simulink model "Quadruped_view"  (R2026a)
settings: Solver=ode23tb  StopTime=50
values from neighbouring files (symbols this model uses):
  a_amp = 0.03    [initializeRobotParameters.m]
  b_amp = 0.03    [initializeRobotParameters.m]
  dTheta = 20*pi/180    (= 0.349065850399)    [initializeRobotParameters.m]
  friction_force_max = mu_static * normal_force_max    [initializeRobotParameters.m]
  g = -9.81    [initializeRobotParameters.m]
  h_final = 0.2    [initializeRobotParameters.m]
  hip_eq_angle = 0    [initializeRobotParameters.m]
  init_ang_FL = d2r * quadrupedInverseKinematics(init_foot_disp_x,-init_body_height,l1,l2)    [initializeRobotParameters.m]
  init_ang_FR = init_ang_FL    [initializeRobotParameters.m]
  init_ang_RL = init_ang_FL    [initializeRobotParameters.m]
  init_ang_RR = init_ang_FL    [initializeRobotParameters.m]
  knee_eq_angle = 0    [initializeRobotParameters.m]
  l1 = 0.1422    [initializeRobotParameters.m]
  l2 = 0.115    [initializeRobotParameters.m]
  L_back = 0.305    [initializeRobotParameters.m]
  M = 1.318    [initializeRobotParameters.m]
  m1 = 0.17824    [initializeRobotParameters.m]
  m2 = 0.03558    [initializeRobotParameters.m]
  normal_force_max = ((M+4*m1+4*m2)*abs(g))/4    [initializeRobotParameters.m]
  period = 0.8    [initializeRobotParameters.m]
  pitch_max = 10 * d2r    (= 0.174532925199)    [initializeRobotParameters.m]
  q_hip_max = -30 * d2r    (= -0.523598775598)    [initializeRobotParameters.m]
  q_hip_min = -120 * d2r    (= -2.09439510239)    [initializeRobotParameters.m]
  q_knee_max = 140 * d2r    (= 2.44346095279)    [initializeRobotParameters.m]
  q_knee_min = 60 * d2r    (= 1.0471975512)    [initializeRobotParameters.m]
  roll_max = 10 * d2r    (= 0.174532925199)    [initializeRobotParameters.m]
  Tf = 10    [initializeRobotParameters.m]
  torso_dim = [L_back 0.04875 0.152]    [initializeRobotParameters.m]
  Tp = 0.15    [initializeRobotParameters.m]
  Ts = 0.025    [initializeRobotParameters.m]
  vx_max = 2.5    [initializeRobotParameters.m]
  vy_max = 2.5    [initializeRobotParameters.m]
  vz_max = 2.5    [initializeRobotParameters.m]
  w_max = 2*pi*60/60    (= 6.28318530718)    [initializeRobotParameters.m]
  y_init = init_body_height + foot_height    [initializeRobotParameters.m]
  y_max = l1*cos(q_hip_max) + l2*cos(q_hip_max+q_knee_min)    [initializeRobotParameters.m]
  y_min = 0.5    [initializeRobotParameters.m]
  yaw_max = 20 * d2r    (= 0.349065850399)    [initializeRobotParameters.m]
  z_max = 0.5    [initializeRobotParameters.m]
undefined symbols (not defined in the file or in its folder): Extr_Data_LinkEndHole, Extr_Data_Mesh, ground, joint, X, Y, Z
libraries: sm_lib x118, nesl_utility x54, simulink x4
(part 2 of 5)

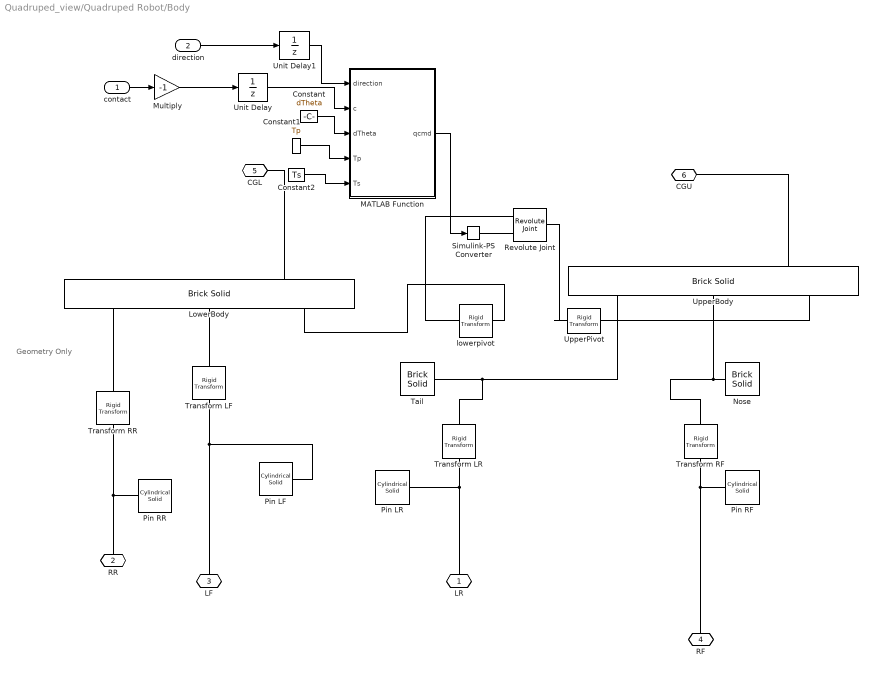
== system Quadruped_view/Quadruped Robot/Body ==
  note: Geometry Only
  contact : Inport
  direction : Inport  Port=2
  Constant : Constant  Value=dTheta
  Constant1 : Constant  Value=Tp
  Constant2 : Constant  Value=Ts
  LowerBody : sm_lib/Body Elements/Brick Solid  BrickDimensions=torso_dim  BrickDimensionsUnits=m  ExportEntireGeometry=off  InertiaType=Custom  BasedOnType=Density  Density=1000  DensityUnits=kg/m^3  Mass=M  MassUnits=kg  CenterOfMass=torso_COM  CenterOfMassUnits=m  MomentsOfInertia=torso_MOI  MomentsOfInertiaUnits=kg*m^2  ProductsOfInertia=torso_POI  ProductsOfInertiaUnits=kg*m^2  GraphicType=FromGeometry  MarkerShape=Sphere  MarkerSize=10  GraphicVisPropType=SimpleVisualProperties  GraphicDiffuseColor=[164 184 200]/255  GraphicOpacity=1.0  GraphicSpecularColor=[0.5 0.5 0.5 1.0]  GraphicAmbientColor=[0.15 0.15 0.15 1.0]  GraphicEmissiveColor=[0.0 0.0 0.0 1.0]  GraphicShininess=75  DoExposeReferenceFrame=on  SerializedFrames=<Frames><Frame><Id>Frame1</Id><Value><Name>B</Name><Origin><Source>GeometricFeature</Source><FeatureName>-x surface</FeatureName></Origin><PrimaryAxis><DefinedDirection>+Z</DefinedDirection><Source>ReferenceFrame</Source><SourceDirection>+Z</SourceDirection><FeatureName></FeatureName></PrimaryAxis><SecondaryAxis><DefinedDirection>+X</DefinedDirection><Source>ReferenceFrame</Source><SourceDirection>+X</SourceDirection><FeatureName></FeatureName></SecondaryAxis></Value></Frame><Frame><Id>Frame2</Id><Value><Name>F</Name><Origin><Source>GeometricFeature</Source><FeatureName>+x surface</FeatureName></Origin><PrimaryAxis><DefinedDirection>+Z</DefinedDirection><Source>ReferenceFrame</Source><SourceDirection>+Z</SourceDirection><FeatureName></FeatureName></PrimaryAxis><SecondaryAxis><DefinedDirection>+X</DefinedDirection><Source>ReferenceFrame</Source><SourceDirection>+X</SourceDirection><FeatureName></FeatureName></SecondaryAxis></Value></Frame><Frame><Id>Frame3</Id><Value><Name>torso_COM</Name><Origin><Source>CenterOfMassFrame</Source><FeatureName></FeatureName></Origin><PrimaryAxis><DefinedDirection>+Z</DefinedDirection><Source>ReferenceFrame</Source><SourceDirection>+Z</SourceDirection><FeatureName></FeatureName></PrimaryAxis><SecondaryAxis><DefinedDirection>+X</DefinedDirection><Source>ReferenceFrame</Source><SourceDirection>+X</SourceDirection><FeatureName></FeatureName></SecondaryAxis></Value></Frame><Frame><Id>Frame4</Id><Value><Name>Origin</Name><Origin><Source>ReferenceFrame</Source><FeatureName></FeatureName></Origin><PrimaryAxis><DefinedDirection>+Z</DefinedDirection><Source>ReferenceFrame</Source><SourceDirection>+Z</SourceDirection><FeatureName></FeatureName></PrimaryAxis><SecondaryAxis><DefinedDirection>+X</DefinedDirection><Source>ReferenceFrame</Source><SourceDirection>+X</SourceDirection><FeatureName></FeatureName></SecondaryAxis></Value></Frame></Frames>
  MATLAB Function : MATLAB Function  TreatAsAtomicUnit=on
  Multiply : Gain  Gain=-1
  Nose : sm_lib/Body Elements/Brick Solid  BrickDimensions=[0.05 0.1 0.1]*L_back  BrickDimensionsUnits=m  ExportEntireGeometry=off  InertiaType=CalculateFromGeometry  BasedOnType=Density  Density=0  DensityUnits=kg/m^3  Mass=1  MassUnits=kg  CenterOfMass=[0 0 0]  CenterOfMassUnits=m  MomentsOfInertia=[1 1 1]  MomentsOfInertiaUnits=kg*m^2  ProductsOfInertia=[1 1 1]  ProductsOfInertiaUnits=kg*m^2  GraphicType=FromGeometry  MarkerShape=Sphere  MarkerSize=10  GraphicVisPropType=SimpleVisualProperties  GraphicDiffuseColor=[164 184 200]/255  GraphicOpacity=1.0  GraphicSpecularColor=[0.5 0.5 0.5 1.0]  GraphicAmbientColor=[0.15 0.15 0.15 1.0]  GraphicEmissiveColor=[0.0 0.0 0.0 1.0]  GraphicShininess=75  DoExposeReferenceFrame=off  SerializedFrames=<Frames><Frame><Id>Frame1</Id><Value><Name>B</Name><Origin><Source>GeometricFeature</Source><FeatureName>-x surface</FeatureName></Origin><PrimaryAxis><DefinedDirection>+Z</DefinedDirection><Source>ReferenceFrame</Source><SourceDirection>+Z</SourceDirection><FeatureName></FeatureName></PrimaryAxis><SecondaryAxis><DefinedDirection>+X</DefinedDirection><Source>ReferenceFrame</Source><SourceDirection>+X</SourceDirection><FeatureName></FeatureName></SecondaryAxis></Value></Frame></Frames>
  Pin LF : sm_lib/Body Elements/Cylindrical Solid  CylinderRadius=0.025*l1  CylinderRadiusUnits=m  CylinderLength=0.1*l1  CylinderLengthUnits=m  ExportEntireGeometry=off  InertiaType=CalculateFromGeometry  BasedOnType=Density  Density=0  DensityUnits=kg/m^3  Mass=1  MassUnits=kg  CenterOfMass=[0 0 0]  CenterOfMassUnits=m  MomentsOfInertia=[1 1 1]  MomentsOfInertiaUnits=kg*m^2  ProductsOfInertia=[1 1 1]  ProductsOfInertiaUnits=kg*m^2  GraphicType=FromGeometry  MarkerShape=Sphere  MarkerSize=10  GraphicVisPropType=SimpleVisualProperties  GraphicDiffuseColor=[164 184 200]/255  GraphicOpacity=1.0  GraphicSpecularColor=[0.5 0.5 0.5 1.0]  GraphicAmbientColor=[0.15 0.15 0.15 1.0]  GraphicEmissiveColor=[0.0 0.0 0.0 1.0]  GraphicShininess=75  DoExposeReferenceFrame=off  SerializedFrames=<Frames><Frame><Id>Frame1</Id><Value><Name>F</Name><Origin><Source>GeometricFeature</Source><FeatureName>top surface</FeatureName></Origin><PrimaryAxis><DefinedDirection>+Z</DefinedDirection><Source>ReferenceFrame</Source><SourceDirection>+Z</SourceDirection><FeatureName></FeatureName></PrimaryAxis><SecondaryAxis><DefinedDirection>+X</DefinedDirection><Source>ReferenceFrame</Source><SourceDirection>+X</SourceDirection><FeatureName></FeatureName></SecondaryAxis></Value></Frame><Frame><Id>Frame2</Id><Value><Name>B</Name><Origin><Source>GeometricFeature</Source><FeatureName>bottom surface</FeatureName></Origin><PrimaryAxis><DefinedDirection>+Z</DefinedDirection><Source>ReferenceFrame</Source><SourceDirection>+Z</SourceDirection><FeatureName></FeatureName></PrimaryAxis><SecondaryAxis><DefinedDirection>+X</DefinedDirection><Source>ReferenceFrame</Source><SourceDirection>+X</SourceDirection><FeatureName></FeatureName></SecondaryAxis></Value></Frame></Frames>
  Pin LR : sm_lib/Body Elements/Cylindrical Solid  CylinderRadius=0.025*l1  CylinderRadiusUnits=m  CylinderLength=0.1*l1  CylinderLengthUnits=m  ExportEntireGeometry=off  InertiaType=CalculateFromGeometry  BasedOnType=Density  Density=0  DensityUnits=kg/m^3  Mass=1  MassUnits=kg  CenterOfMass=[0 0 0]  CenterOfMassUnits=m  MomentsOfInertia=[1 1 1]  MomentsOfInertiaUnits=kg*m^2  ProductsOfInertia=[1 1 1]  ProductsOfInertiaUnits=kg*m^2  GraphicType=FromGeometry  MarkerShape=Sphere  MarkerSize=10  GraphicVisPropType=SimpleVisualProperties  GraphicDiffuseColor=[164 184 200]/255  GraphicOpacity=1.0  GraphicSpecularColor=[0.5 0.5 0.5 1.0]  GraphicAmbientColor=[0.15 0.15 0.15 1.0]  GraphicEmissiveColor=[0.0 0.0 0.0 1.0]  GraphicShininess=75  DoExposeReferenceFrame=off  SerializedFrames=<Frames><Frame><Id>Frame1</Id><Value><Name>F</Name><Origin><Source>GeometricFeature</Source><FeatureName>top surface</FeatureName></Origin><PrimaryAxis><DefinedDirection>+Z</DefinedDirection><Source>ReferenceFrame</Source><SourceDirection>+Z</SourceDirection><FeatureName></FeatureName></PrimaryAxis><SecondaryAxis><DefinedDirection>+X</DefinedDirection><Source>ReferenceFrame</Source><SourceDirection>+X</SourceDirection><FeatureName></FeatureName></SecondaryAxis></Value></Frame><Frame><Id>Frame2</Id><Value><Name>B</Name><Origin><Source>GeometricFeature</Source><FeatureName>bottom surface</FeatureName></Origin><PrimaryAxis><DefinedDirection>+Z</DefinedDirection><Source>ReferenceFrame</Source><SourceDirection>+Z</SourceDirection><FeatureName></FeatureName></PrimaryAxis><SecondaryAxis><DefinedDirection>+X</DefinedDirection><Source>ReferenceFrame</Source><SourceDirection>+X</SourceDirection><FeatureName></FeatureName></SecondaryAxis></Value></Frame></Frames>
  Pin RF : sm_lib/Body Elements/Cylindrical Solid  CylinderRadius=0.025*l1  CylinderRadiusUnits=m  CylinderLength=0.1*l1  CylinderLengthUnits=m  ExportEntireGeometry=off  InertiaType=CalculateFromGeometry  BasedOnType=Density  Density=0  DensityUnits=kg/m^3  Mass=1  MassUnits=kg  CenterOfMass=[0 0 0]  CenterOfMassUnits=m  MomentsOfInertia=[1 1 1]  MomentsOfInertiaUnits=kg*m^2  ProductsOfInertia=[1 1 1]  ProductsOfInertiaUnits=kg*m^2  GraphicType=FromGeometry  MarkerShape=Sphere  MarkerSize=10  GraphicVisPropType=SimpleVisualProperties  GraphicDiffuseColor=[164 184 200]/255  GraphicOpacity=1.0  GraphicSpecularColor=[0.5 0.5 0.5 1.0]  GraphicAmbientColor=[0.15 0.15 0.15 1.0]  GraphicEmissiveColor=[0.0 0.0 0.0 1.0]  GraphicShininess=75  DoExposeReferenceFrame=off  SerializedFrames=<Frames><Frame><Id>Frame1</Id><Value><Name>F</Name><Origin><Source>GeometricFeature</Source><FeatureName>top surface</FeatureName></Origin><PrimaryAxis><DefinedDirection>+Z</DefinedDirection><Source>ReferenceFrame</Source><SourceDirection>+Z</SourceDirection><FeatureName></FeatureName></PrimaryAxis><SecondaryAxis><DefinedDirection>+X</DefinedDirection><Source>ReferenceFrame</Source><SourceDirection>+X</SourceDirection><FeatureName></FeatureName></SecondaryAxis></Value></Frame><Frame><Id>Frame2</Id><Value><Name>B</Name><Origin><Source>GeometricFeature</Source><FeatureName>bottom surface</FeatureName></Origin><PrimaryAxis><DefinedDirection>+Z</DefinedDirection><Source>ReferenceFrame</Source><SourceDirection>+Z</SourceDirection><FeatureName></FeatureName></PrimaryAxis><SecondaryAxis><DefinedDirection>+X</DefinedDirection><Source>ReferenceFrame</Source><SourceDirection>+X</SourceDirection><FeatureName></FeatureName></SecondaryAxis></Value></Frame></Frames>
  Pin RR : sm_lib/Body Elements/Cylindrical Solid  CylinderRadius=0.025*l1  CylinderRadiusUnits=m  CylinderLength=0.1*l1  CylinderLengthUnits=m  ExportEntireGeometry=off  InertiaType=CalculateFromGeometry  BasedOnType=Density  Density=0  DensityUnits=kg/m^3  Mass=1  MassUnits=kg  CenterOfMass=[0 0 0]  CenterOfMassUnits=m  MomentsOfInertia=[1 1 1]  MomentsOfInertiaUnits=kg*m^2  ProductsOfInertia=[1 1 1]  ProductsOfInertiaUnits=kg*m^2  GraphicType=FromGeometry  MarkerShape=Sphere  MarkerSize=10  GraphicVisPropType=SimpleVisualProperties  GraphicDiffuseColor=[164 184 200]/255  GraphicOpacity=1.0  GraphicSpecularColor=[0.5 0.5 0.5 1.0]  GraphicAmbientColor=[0.15 0.15 0.15 1.0]  GraphicEmissiveColor=[0.0 0.0 0.0 1.0]  GraphicShininess=75  DoExposeReferenceFrame=off  SerializedFrames=<Frames><Frame><Id>Frame1</Id><Value><Name>F</Name><Origin><Source>GeometricFeature</Source><FeatureName>top surface</FeatureName></Origin><PrimaryAxis><DefinedDirection>+Z</DefinedDirection><Source>ReferenceFrame</Source><SourceDirection>+Z</SourceDirection><FeatureName></FeatureName></PrimaryAxis><SecondaryAxis><DefinedDirection>+X</DefinedDirection><Source>ReferenceFrame</Source><SourceDirection>+X</SourceDirection><FeatureName></FeatureName></SecondaryAxis></Value></Frame><Frame><Id>Frame2</Id><Value><Name>B</Name><Origin><Source>GeometricFeature</Source><FeatureName>bottom surface</FeatureName></Origin><PrimaryAxis><DefinedDirection>+Z</DefinedDirection><Source>ReferenceFrame</Source><SourceDirection>+Z</SourceDirection><FeatureName></FeatureName></PrimaryAxis><SecondaryAxis><DefinedDirection>+X</DefinedDirection><Source>ReferenceFrame</Source><SourceDirection>+X</SourceDirection><FeatureName></FeatureName></SecondaryAxis></Value></Frame></Frames>
  Revolute Joint : sm_lib/Joints/Revolute Joint  JointMode=Normal  CompositeWrenchDir=FollowerOnBase  CompositeWrenchFrame=BaseFrame  SenseConstraintForce=off  SenseConstraintTorque=off  SenseTotalForce=off  SenseTotalTorque=off  PositionTargetSpecify=off  PositionTargetPriority=High  PositionTargetValue=0  PositionTargetValueUnits=deg  VelocityTargetSpecify=off  VelocityTargetPriority=High  VelocityTargetValue=0  VelocityTargetValueUnits=deg/s  EquilibriumPosition=0  EquilibriumPositionUnits=deg  SpringStiffness=0  SpringStiffnessUnits=N*m/deg  DampingCoefficient=0  DampingCoefficientUnits=N*m/(deg/s)  LowerLimitSpecify=off  LowerLimitBound=-90  LowerLimitBoundUnits=deg  LowerLimitStiffness=1e4  LowerLimitStiffnessUnits=N*m/deg  LowerLimitDamping=10  LowerLimitDampingUnits=N*m/(deg/s)  LowerLimitTransitionRegionWidth=0.1  LowerLimitTransitionRegionWidthUnits=deg  UpperLimitSpecify=off  UpperLimitBound=90  UpperLimitBoundUnits=deg  UpperLimitStiffness=1e4  UpperLimitStiffnessUnits=N*m/deg  UpperLimitDamping=10  UpperLimitDampingUnits=N*m/(deg/s)  UpperLimitTransitionRegionWidth=0.1  UpperLimitTransitionRegionWidthUnits=deg  TorqueActuationMode=ComputedTorque  MotionActuationMode=InputMotion  SensePosition=off  SenseVelocity=off  SenseAcceleration=off  SenseTorqueForce=off  SenseLowerLimitTorqueForce=off  SenseUpperLimitTorqueForce=off
  Simulink-PS Converter : nesl_utility/Simulink-PS Converter  PhysicalDomain=network_engine_domain  SubClassName=ps_input  LeftPortType=input  RightPortType=output  PseudoPeriodic=off  Frequencies=[]  NoiseDistribution=none  NoiseParameters=[]  Unit=1  AffineConversion=off  FilteringAndDerivatives=filter  SimscapeFilterOrder=2  InputFilterTimeConstant=0.001  UdotUserProvided=0
  Tail : sm_lib/Body Elements/Brick Solid  BrickDimensions=[0.05 0.1 0.1]*L_back  BrickDimensionsUnits=m  ExportEntireGeometry=off  InertiaType=CalculateFromGeometry  BasedOnType=Density  Density=0  DensityUnits=kg/m^3  Mass=1  MassUnits=kg  CenterOfMass=[0 0 0]  CenterOfMassUnits=m  MomentsOfInertia=[1 1 1]  MomentsOfInertiaUnits=kg*m^2  ProductsOfInertia=[1 1 1]  ProductsOfInertiaUnits=kg*m^2  GraphicType=FromGeometry  MarkerShape=Sphere  MarkerSize=10  GraphicVisPropType=SimpleVisualProperties  GraphicDiffuseColor=[164 184 200]/255  GraphicOpacity=1.0  GraphicSpecularColor=[0.5 0.5 0.5 1.0]  GraphicAmbientColor=[0.15 0.15 0.15 1.0]  GraphicEmissiveColor=[0.0 0.0 0.0 1.0]  GraphicShininess=75  DoExposeReferenceFrame=off  SerializedFrames=<Frames><Frame><Id>Frame1</Id><Value><Name>F</Name><Origin><Source>GeometricFeature</Source><FeatureName>+x surface</FeatureName></Origin><PrimaryAxis><DefinedDirection>+Z</DefinedDirection><Source>ReferenceFrame</Source><SourceDirection>+Z</SourceDirection><FeatureName></FeatureName></PrimaryAxis><SecondaryAxis><DefinedDirection>+X</DefinedDirection><Source>ReferenceFrame</Source><SourceDirection>+X</SourceDirection><FeatureName></FeatureName></SecondaryAxis></Value></Frame></Frames>
  Transform LF : sm_lib/Frames and Transforms/Rigid Transform  RotationMethod=None  FollAlignAxisA=+X  BaseAlignAxisA=+Y  FollAlignAxisB=+Y  BaseAlignAxisB=+Z  RotationStandardAxis=+Z  RotationAngle=0.0  RotationAngleUnits=deg  RotationArbitraryAxis=[0 0 1]  RotationSequenceAxes=FollowerAxes  RotationSequence=XYX  RotationSequenceAngles=[0 0 0]  RotationSequenceAnglesUnits=deg  RotationMatrix=[1 0 0; 0 1 0; 0 0 1]  Quaternion=[1 0 0 0]  TranslationMethod=Cartesian  TranslationCartesianOffset=[0 -torso_dim(2)/2 torso_dim(3)/2]  TranslationCartesianOffsetUnits=m  TranslationStandardAxis=+Z  TranslationStandardOffset=torso_dim(3)/2  TranslationStandardOffsetUnits=m  TranslationROffset=0  TranslationROffsetUnits=m  TranslationThetaOffset=0  TranslationThetaOffsetUnits=deg  TranslationZOffset=0  TranslationZOffsetUnits=m
  Transform LR : sm_lib/Frames and Transforms/Rigid Transform  RotationMethod=None  FollAlignAxisA=+X  BaseAlignAxisA=+Y  FollAlignAxisB=+Y  BaseAlignAxisB=+Z  RotationStandardAxis=+Z  RotationAngle=0.0  RotationAngleUnits=deg  RotationArbitraryAxis=[0 0 1]  RotationSequenceAxes=FollowerAxes  RotationSequence=XYX  RotationSequenceAngles=[0 0 0]  RotationSequenceAnglesUnits=deg  RotationMatrix=[1 0 0; 0 1 0; 0 0 1]  Quaternion=[1 0 0 0]  TranslationMethod=Cartesian  TranslationCartesianOffset=[0 torso_dim(2)/2 torso_dim(3)/2]  TranslationCartesianOffsetUnits=m  TranslationStandardAxis=+Y  TranslationStandardOffset=-torso_dim(2)/2  TranslationStandardOffsetUnits=m  TranslationROffset=0  TranslationROffsetUnits=m  TranslationThetaOffset=0  TranslationThetaOffsetUnits=deg  TranslationZOffset=0  TranslationZOffsetUnits=m
  Transform RF : sm_lib/Frames and Transforms/Rigid Transform  RotationMethod=None  FollAlignAxisA=+X  BaseAlignAxisA=+Y  FollAlignAxisB=+Y  BaseAlignAxisB=+Z  RotationStandardAxis=+Z  RotationAngle=0.0  RotationAngleUnits=deg  RotationArbitraryAxis=[0 0 1]  RotationSequenceAxes=FollowerAxes  RotationSequence=XYX  RotationSequenceAngles=[0 0 0]  RotationSequenceAnglesUnits=deg  RotationMatrix=[1 0 0; 0 1 0; 0 0 1]  Quaternion=[1 0 0 0]  TranslationMethod=Cartesian  TranslationCartesianOffset=[0 -torso_dim(2)/2 torso_dim(3)/2]  TranslationCartesianOffsetUnits=m  TranslationStandardAxis=+Z  TranslationStandardOffset=torso_dim(3)/2  TranslationStandardOffsetUnits=m  TranslationROffset=0  TranslationROffsetUnits=m  TranslationThetaOffset=0  TranslationThetaOffsetUnits=deg  TranslationZOffset=0  TranslationZOffsetUnits=m
  Transform RR : sm_lib/Frames and Transforms/Rigid Transform  RotationMethod=None  FollAlignAxisA=+X  BaseAlignAxisA=+Y  FollAlignAxisB=+Y  BaseAlignAxisB=+Z  RotationStandardAxis=+Z  RotationAngle=0.0  RotationAngleUnits=deg  RotationArbitraryAxis=[0 0 1]  RotationSequenceAxes=FollowerAxes  RotationSequence=XYX  RotationSequenceAngles=[0 0 0]  RotationSequenceAnglesUnits=deg  RotationMatrix=[1 0 0; 0 1 0; 0 0 1]  Quaternion=[1 0 0 0]  TranslationMethod=Cartesian  TranslationCartesianOffset=[0 torso_dim(2)/2 torso_dim(3)/2]  TranslationCartesianOffsetUnits=m  TranslationStandardAxis=+Z  TranslationStandardOffset=torso_dim(3)/2  TranslationStandardOffsetUnits=m  TranslationROffset=0  TranslationROffsetUnits=m  TranslationThetaOffset=0  TranslationThetaOffsetUnits=deg  TranslationZOffset=0  TranslationZOffsetUnits=m
  Unit Delay : UnitDelay  SampleTime=Ts
  Unit Delay1 : UnitDelay  SampleTime=0.6
  UpperBody : sm_lib/Body Elements/Brick Solid  BrickDimensions=torso_dim  BrickDimensionsUnits=m  ExportEntireGeometry=off  InertiaType=Custom  BasedOnType=Density  Density=1000  DensityUnits=kg/m^3  Mass=M  MassUnits=kg  CenterOfMass=torso_COM  CenterOfMassUnits=m  MomentsOfInertia=torso_MOI  MomentsOfInertiaUnits=kg*m^2  ProductsOfInertia=torso_POI  ProductsOfInertiaUnits=kg*m^2  GraphicType=FromGeometry  MarkerShape=Sphere  MarkerSize=10  GraphicVisPropType=SimpleVisualProperties  GraphicDiffuseColor=[164 184 200]/255  GraphicOpacity=1.0  GraphicSpecularColor=[0.5 0.5 0.5 1.0]  GraphicAmbientColor=[0.15 0.15 0.15 1.0]  GraphicEmissiveColor=[0.0 0.0 0.0 1.0]  GraphicShininess=75  DoExposeReferenceFrame=on  SerializedFrames=<Frames><Frame><Id>Frame1</Id><Value><Name>B</Name><Origin><Source>GeometricFeature</Source><FeatureName>-x surface</FeatureName></Origin><PrimaryAxis><DefinedDirection>+Z</DefinedDirection><Source>ReferenceFrame</Source><SourceDirection>+Z</SourceDirection><FeatureName></FeatureName></PrimaryAxis><SecondaryAxis><DefinedDirection>+X</DefinedDirection><Source>ReferenceFrame</Source><SourceDirection>+X</SourceDirection><FeatureName></FeatureName></SecondaryAxis></Value></Frame><Frame><Id>Frame2</Id><Value><Name>F</Name><Origin><Source>GeometricFeature</Source><FeatureName>+x surface</FeatureName></Origin><PrimaryAxis><DefinedDirection>+Z</DefinedDirection><Source>ReferenceFrame</Source><SourceDirection>+Z</SourceDirection><FeatureName></FeatureName></PrimaryAxis><SecondaryAxis><DefinedDirection>+X</DefinedDirection><Source>ReferenceFrame</Source><SourceDirection>+X</SourceDirection><FeatureName></FeatureName></SecondaryAxis></Value></Frame><Frame><Id>Frame3</Id><Value><Name>torso_COM</Name><Origin><Source>CenterOfMassFrame</Source><FeatureName></FeatureName></Origin><PrimaryAxis><DefinedDirection>+Z</DefinedDirection><Source>ReferenceFrame</Source><SourceDirection>+Z</SourceDirection><FeatureName></FeatureName></PrimaryAxis><SecondaryAxis><DefinedDirection>+X</DefinedDirection><Source>ReferenceFrame</Source><SourceDirection>+X</SourceDirection><FeatureName></FeatureName></SecondaryAxis></Value></Frame><Frame><Id>Frame4</Id><Value><Name>Origin</Name><Origin><Source>ReferenceFrame</Source><FeatureName></FeatureName></Origin><PrimaryAxis><DefinedDirection>+Z</DefinedDirection><Source>ReferenceFrame</Source><SourceDirection>+Z</SourceDirection><FeatureName></FeatureName></PrimaryAxis><SecondaryAxis><DefinedDirection>+X</DefinedDirection><Source>ReferenceFrame</Source><SourceDirection>+X</SourceDirection><FeatureName></FeatureName></SecondaryAxis></Value></Frame></Frames>
  UpperPivot : sm_lib/Frames and Transforms/Rigid Transform  RotationMethod=StandardAxis  FollAlignAxisA=+X  BaseAlignAxisA=+Y  FollAlignAxisB=+Y  BaseAlignAxisB=+Z  RotationStandardAxis=+X  RotationAngle=-90  RotationAngleUnits=deg  RotationArbitraryAxis=[0 0 1]  RotationSequenceAxes=FollowerAxes  RotationSequence=XYX  RotationSequenceAngles=[0 0 0]  RotationSequenceAnglesUnits=deg  RotationMatrix=[1 0 0;0 1 0;0 0 1]  Quaternion=[1 0 0 0]  TranslationMethod=Cartesian  TranslationCartesianOffset=[0 0 -torso_dim(2)/2]  TranslationCartesianOffsetUnits=m  TranslationStandardAxis=+Z  TranslationStandardOffset=0  TranslationStandardOffsetUnits=m  TranslationROffset=0  TranslationROffsetUnits=m  TranslationThetaOffset=0  TranslationThetaOffsetUnits=deg  TranslationZOffset=0  TranslationZOffsetUnits=m
  lowerpivot : sm_lib/Frames and Transforms/Rigid Transform  RotationMethod=StandardAxis  FollAlignAxisA=+X  BaseAlignAxisA=+Y  FollAlignAxisB=+Y  BaseAlignAxisB=+Z  RotationStandardAxis=+X  RotationAngle=-90  RotationAngleUnits=deg  RotationArbitraryAxis=[0 0 1]  RotationSequenceAxes=FollowerAxes  RotationSequence=XYX  RotationSequenceAngles=[0 0 0]  RotationSequenceAnglesUnits=deg  RotationMatrix=[1 0 0;0 1 0;0 0 1]  Quaternion=[1 0 0 0]  TranslationMethod=Cartesian  TranslationCartesianOffset=[0 0 torso_dim(2)/2]  TranslationCartesianOffsetUnits=m  TranslationStandardAxis=+Z  TranslationStandardOffset=0  TranslationStandardOffsetUnits=m  TranslationROffset=0  TranslationROffsetUnits=m  TranslationThetaOffset=0  TranslationThetaOffsetUnits=deg  TranslationZOffset=0  TranslationZOffsetUnits=m
  LR : PMIOPort  Side=Left
  RR : PMIOPort  Port=2  Side=Left
  LF : PMIOPort  Port=3  Side=Left
  RF : PMIOPort  Port=4  Side=Left
  CGL : PMIOPort  Port=5  Side=Left
  CGU : PMIOPort  Port=6  Side=Left
  wires:
  contact/1 -> Multiply/1
  Multiply/1 -> Unit Delay/1
  MATLAB Function/1(qcmd) -> Simulink-PS Converter/1
  Constant/1 -> MATLAB Function/3(dTheta)
  Constant1/1 -> MATLAB Function/4(Tp)
  Constant2/1 -> MATLAB Function/5(Ts)
  Unit Delay/1 -> MATLAB Function/2(c)
  direction/1 -> Unit Delay1/1
  Unit Delay1/1 -> MATLAB Function/1(direction)
  connections:
  Pin RF/RConn1 -- RF/RConn1 -- Transform RF/RConn1
  Transform RF/LConn1 -- Nose/LConn1 -- UpperBody/LConn2
  UpperBody/LConn1 -- Transform LR/RConn1 -- Tail/LConn1
  Transform LR/LConn1 -- Pin LR/LConn1 -- LR/RConn1
  Transform RR/RConn1 -- Pin RR/RConn1 -- RR/RConn1
  LowerBody/LConn1 -- Transform RR/LConn1
  Transform LF/LConn1 -- Pin LF/LConn1 -- LF/RConn1
  LowerBody/LConn2 -- Transform LF/RConn1
  LowerBody/RConn2 -- CGL/RConn1
  UpperBody/RConn2 -- CGU/RConn1
  lowerpivot/RConn1 -- LowerBody/LConn3
  lowerpivot/LConn1 -- Revolute Joint/LConn1
  UpperBody/LConn3 -- UpperPivot/RConn1
  UpperPivot/LConn1 -- Revolute Joint/RConn1
  Simulink-PS Converter/RConn1 -- Revolute Joint/LConn2

== system Quadruped_view/Quadruped Robot/Floor ==
  Floor : sm_lib/Body Elements/Brick Solid  BrickDimensions=[100 0.05 1]  BrickDimensionsUnits=m  ExportEntireGeometry=on  InertiaType=CalculateFromGeometry  BasedOnType=Density  Density=1000  DensityUnits=kg/m^3  Mass=1  MassUnits=kg  CenterOfMass=[0 0 0]  CenterOfMassUnits=m  MomentsOfInertia=[1 1 1]  MomentsOfInertiaUnits=kg*m^2  ProductsOfInertia=[1 1 1]  ProductsOfInertiaUnits=kg*m^2  GraphicType=FromGeometry  MarkerShape=Sphere  MarkerSize=10  GraphicVisPropType=SimpleVisualProperties  GraphicDiffuseColor=[0.5 0.5 0.5]  GraphicOpacity=1.0  GraphicSpecularColor=[0.5 0.5 0.5 1.0]  GraphicAmbientColor=[0.15 0.15 0.15 1.0]  GraphicEmissiveColor=[0.0 0.0 0.0 1.0]  GraphicShininess=75  DoExposeReferenceFrame=on  SerializedFrames=<Frames/>
  Mechanism Configuration : sm_lib/Utilities/Mechanism Configuration  UniformGravity=Constant  GravityVector=[0 g 0]  GravityVectorUnits=m/s^2  LinearizationDelta=0.001  JointModeTransitionNonlinearIterations=2
  Mesh : sm_lib/Body Elements/Extruded Solid  ExtrusionType=General  PolygonNumSides=3  PolygonOuterRadius=1  PolygonOuterRadiusUnits=m  ExportEntireGeometry=off  ExtrusionCrossSection=Extr_Data_Mesh(100,1,100,1,0.9,0.9)  ExtrusionCrossSectionUnits=m  ExportConvexHullGeometry=off  ExtrusionLength=0.055  ExtrusionLengthUnits=m  InertiaType=CalculateFromGeometry  BasedOnType=Density  Density=1000  DensityUnits=kg/m^3  Mass=1  MassUnits=kg  CenterOfMass=[0 0 0]  CenterOfMassUnits=m  MomentsOfInertia=[1 1 1]  MomentsOfInertiaUnits=kg*m^2  ProductsOfInertia=[1 1 1]  ProductsOfInertiaUnits=kg*m^2  GraphicType=FromGeometry  MarkerShape=Sphere  MarkerSize=10  GraphicVisPropType=SimpleVisualProperties  GraphicDiffuseColor=[1.0 1.0 1.0]  GraphicOpacity=1.0  GraphicSpecularColor=[0.5 0.5 0.5 1.0]  GraphicAmbientColor=[0.15 0.15 0.15 1.0]  GraphicEmissiveColor=[0.0 0.0 0.0 1.0]  GraphicShininess=75  DoExposeReferenceFrame=on  SerializedFrames=<Frames/>
  Solver Configuration : nesl_utility/Solver Configuration  PhysicalDomain=network_engine_domain  SubClassName=solver  LeftPortType=input  RightPortType=generic  Tones=[]  Harmonics=[]  SimulateNoise=off  Profile=off  UseLocalSampling=off  EnableSwitchedLinearOptims=on  FrequencyDomain=off  UseCCode=off  RelTol=0.001  AbsTol=1e-06  MinStep=1e-09  ToWorkspace=off  RevertToSquareIcSolve=off  NumHomotopyIterations=100  PhasorMode=off  PhasorModeNumHarmonics=1  ConsistencySolver=NEWTON_FTOL  CanonicalOrdering=UNORDERED  OptimizeIntermediates=UNOPTIMIZED  IndexReductionMethod=DerivativeReplacement  DoDC=off  ResidualTolerance=1e-9  ConsistencyTolSource=GLOBAL  ConsistencyAbsTol=0.001  ConsistencyRelTol=0.001  ConsistencyTolFactor=0.001  UseLocalSolver=off  LocalSolverChoice=NE_BACKWARD_EULER_ADVANCER  ResolveIndetEquations=on  FunctionEvalNumThread=1  LocalSolverSampleTime=.001  DoFixedCost=off  MaxNonlinIter=12  MaxModeIter=2  ComputeImpulses=off  ImpulseIterations=2  LinearAlgebra=Sparse  LinearAlgebraNumThread=0  EquationFormulation=NE_TIME_EF  DelaysMemoryBudget=1024  AutomaticFiltering=on  FilteringTimeConstant=0.001  PartitionStorageMethod=AS_NEEDED  PartitionMemoryBudget=1024  PartitionMethod=FAST  MultibodyUseLocalSolver=off  MultibodyLocalSolverChoice=ODE1  MultibodyLocalSolverSampleTime=0.001
  Transform Floor Frame : sm_lib/Frames and Transforms/Rigid Transform  RotationMethod=None  FollAlignAxisA=+X  BaseAlignAxisA=+Y  FollAlignAxisB=+Y  BaseAlignAxisB=+Z  RotationStandardAxis=+X  RotationAngle=-90  RotationAngleUnits=deg  RotationArbitraryAxis=[0 0 1]  RotationSequenceAxes=FollowerAxes  RotationSequence=XYX  RotationSequenceAngles=[0 0 0]  RotationSequenceAnglesUnits=deg  RotationMatrix=[1 0 0; 0 1 0; 0 0 1]  Quaternion=[1 0 0 0]  TranslationMethod=StandardAxis  TranslationCartesianOffset=[0 0 0]  TranslationCartesianOffsetUnits=m  TranslationStandardAxis=-Y  TranslationStandardOffset=0.056/2  TranslationStandardOffsetUnits=m  TranslationROffset=0  TranslationROffsetUnits=m  TranslationThetaOffset=0  TranslationThetaOffsetUnits=deg  TranslationZOffset=0  TranslationZOffsetUnits=m
  Transform Mesh : sm_lib/Frames and Transforms/Rigid Transform  RotationMethod=StandardAxis  FollAlignAxisA=+X  BaseAlignAxisA=+Y  FollAlignAxisB=+Y  BaseAlignAxisB=+Z  RotationStandardAxis=-X  RotationAngle=90  RotationAngleUnits=deg  RotationArbitraryAxis=[0 0 1]  RotationSequenceAxes=FollowerAxes  RotationSequence=XYX  RotationSequenceAngles=[0 0 0]  RotationSequenceAnglesUnits=deg  RotationMatrix=[1 0 0; 0 1 0; 0 0 1]  Quaternion=[1 0 0 0]  TranslationMethod=None  TranslationCartesianOffset=[0 0 0]  TranslationCartesianOffsetUnits=m  TranslationStandardAxis=+Z  TranslationStandardOffset=0  TranslationStandardOffsetUnits=m  TranslationROffset=0  TranslationROffsetUnits=m  TranslationThetaOffset=0  TranslationThetaOffsetUnits=deg  TranslationZOffset=0  TranslationZOffsetUnits=m
  World Frame : sm_lib/Frames and Transforms/World Frame
  FG : PMIOPort  Side=Right
  W : PMIOPort  Port=2  Side=Left
  connections:
  Mesh/RConn1 -- Transform Mesh/RConn1
  Floor/RConn1 -- Transform Mesh/LConn1 -- Transform Floor Frame/RConn1
  Transform Floor Frame/LConn1 -- World Frame/RConn1 -- Solver Configuration/RConn1 -- Mechanism Configuration/RConn1 -- W/RConn1
  FG/RConn1 -- Floor/LConn1

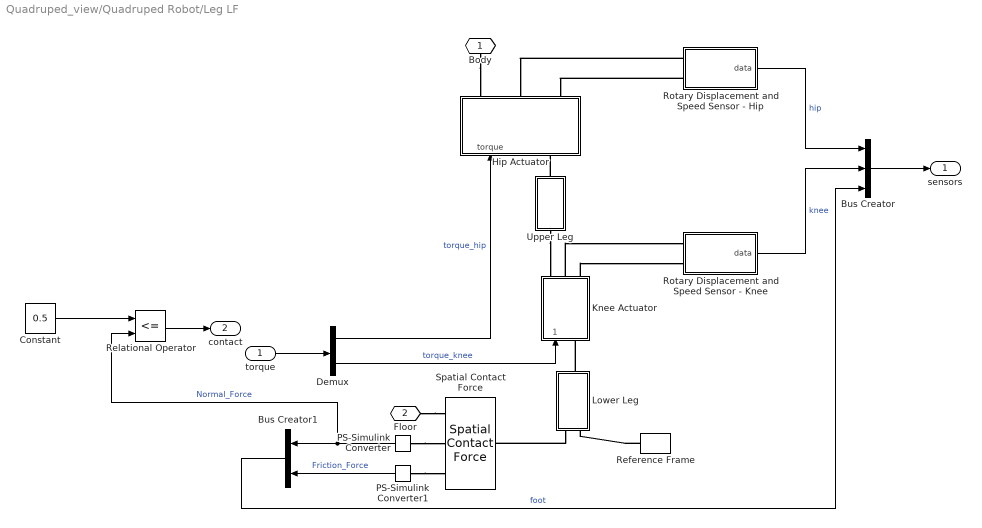
== system Quadruped_view/Quadruped Robot/Leg LF ==
  torque : Inport
  Bus Creator : BusCreator  Inputs=3
  Bus Creator1 : BusCreator  Inputs=2
  Constant : Constant  Value=0.5
  Demux : Demux  Outputs=2
  Hip Actuator : Subsystem
  Knee Actuator : Subsystem
  Lower Leg : Subsystem
  PS-Simulink Converter : nesl_utility/PS-Simulink Converter  PhysicalDomain=network_engine_domain  SubClassName=ps_output  LeftPortType=input  RightPortType=output  PseudoPeriodic=off  Frequencies=[]  VectorFormat=1-D array  Unit=inherit  AffineConversion=off
  PS-Simulink Converter1 : nesl_utility/PS-Simulink Converter  PhysicalDomain=network_engine_domain  SubClassName=ps_output  LeftPortType=input  RightPortType=output  PseudoPeriodic=off  Frequencies=[]  VectorFormat=1-D array  Unit=inherit  AffineConversion=off
  Reference Frame : sm_lib/Frames and Transforms/Reference Frame
  Relational Operator : RelationalOperator  Operator=<=  OutDataTypeStr=boolean  RndMeth=Simplest  InputSameDT=off
  Rotary Displacement and Speed Sensor - Hip : Subsystem
  Rotary Displacement and Speed Sensor - Knee : Subsystem
  Spatial Contact Force : sm_lib/Forces and Torques/Spatial Contact Force  SenseSeparationDistance=off  NormalForceType=SmoothSpringDamper  NormalStiffness=ground.stiffness  NormalStiffnessUnits=N/m  NormalDamping=ground.damping  NormalDampingUnits=N/(m/s)  NormalTransitionRegionWidth=ground.depth/2  NormalTransitionRegionWidthUnits=m  FrictionType=SmoothStickSlip  CoefficientOfStaticFriction=mu_static  CoefficientOfDynamicFriction=mu_kinetic  FrictionalCriticalVelocity=v_thres  FrictionalCriticalVelocityUnits=m/s  SenseContactSignal=off  SensePenetrationDepth=off  SenseNormalVelocity=off  SenseTangentialVelocity=off  SensingForceTorqueDirection=BaseOnFollower  SensingForceTorqueResolutionFrame=ContactFrame  SenseNormalForce=off  SenseNormalForceMagnitude=on  SenseNormalTorque=off  SenseFrictionalForce=off  SenseFrictionalForceMagnitude=on  SenseFrictionalTorque=off  SenseTotalForce=off  SenseTotalTorque=off  SenseContactBaseRotation=off  SenseContactBaseTranslation=off  SenseContactFollowerRotation=off  SenseContactFollowerTranslation=off  ZeroCrossDetectContactStartAndEnd=off
  Upper Leg : Subsystem
  Body : PMIOPort  Side=Left
  Floor : PMIOPort  Tag=PMCPort  Port=2  Side=Right
  sensors : Outport  VectorParamsAs1DForOutWhenUnconnected=off
  contact : Outport  Port=2
  wires:
  Bus Creator/1 -> sensors/1
  Rotary Displacement and Speed Sensor - Knee/1(data) -> Bus Creator/2  "knee"
  Rotary Displacement and Speed Sensor - Hip/1(data) -> Bus Creator/1  "hip"
  Demux/2 -> Knee Actuator/1(torque)  "torque_knee"
  Demux/1 -> Hip Actuator/1(torque)  "torque_hip"
  torque/1 -> Demux/1
  PS-Simulink Converter1/1 -> Bus Creator1/2  "Friction_Force"
  PS-Simulink Converter/1 -> Relational Operator/2, Bus Creator1/1  "Normal_Force"
  Bus Creator1/1 -> Bus Creator/3  "foot"
  Constant/1 -> Relational Operator/1
  Relational Operator/1 -> contact/1
  connections:
  Knee Actuator/RConn3 -- Rotary Displacement and Speed Sensor - Knee/LConn2
  Knee Actuator/RConn2 -- Rotary Displacement and Speed Sensor - Knee/LConn1
  Rotary Displacement and Speed Sensor - Hip/LConn2 -- Hip Actuator/RConn3
  Rotary Displacement and Speed Sensor - Hip/LConn1 -- Hip Actuator/RConn2
  Upper Leg/LConn1 -- Knee Actuator/RConn1
  Upper Leg/RConn1 -- Hip Actuator/LConn1
  Lower Leg/RConn1 -- Knee Actuator/LConn1
  Body/RConn1 -- Hip Actuator/RConn1
  Lower Leg/LConn1 -- Spatial Contact Force/LConn1
  Floor/RConn1 -- Spatial Contact Force/RConn1
  PS-Simulink Converter1/LConn1 -- Spatial Contact Force/RConn3
  PS-Simulink Converter/LConn1 -- Spatial Contact Force/RConn2
  Reference Frame/RConn1 -- Lower Leg/LConn2

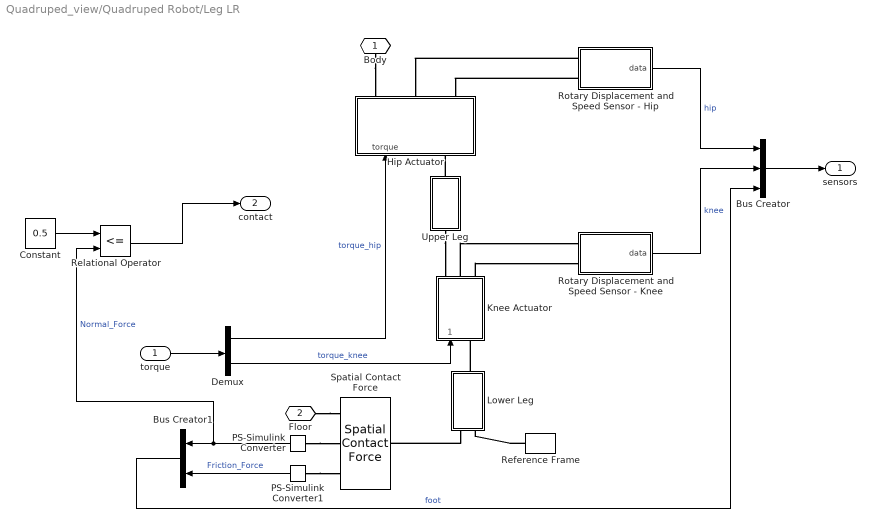
== system Quadruped_view/Quadruped Robot/Leg LR ==
  torque : Inport
  Bus Creator : BusCreator  Inputs=3
  Bus Creator1 : BusCreator  Inputs=2
  Constant : Constant  Value=0.5
  Demux : Demux  Outputs=2
  Hip Actuator : Subsystem
  Knee Actuator : Subsystem
  Lower Leg : Subsystem
  PS-Simulink Converter : nesl_utility/PS-Simulink Converter  PhysicalDomain=network_engine_domain  SubClassName=ps_output  LeftPortType=input  RightPortType=output  PseudoPeriodic=off  Frequencies=[]  VectorFormat=1-D array  Unit=inherit  AffineConversion=off
  PS-Simulink Converter1 : nesl_utility/PS-Simulink Converter  PhysicalDomain=network_engine_domain  SubClassName=ps_output  LeftPortType=input  RightPortType=output  PseudoPeriodic=off  Frequencies=[]  VectorFormat=1-D array  Unit=inherit  AffineConversion=off
  Reference Frame : sm_lib/Frames and Transforms/Reference Frame
  Relational Operator : RelationalOperator  Operator=<=  OutDataTypeStr=boolean  RndMeth=Simplest  InputSameDT=off
  Rotary Displacement and Speed Sensor - Hip : Subsystem
  Rotary Displacement and Speed Sensor - Knee : Subsystem
  Spatial Contact Force : sm_lib/Forces and Torques/Spatial Contact Force  SenseSeparationDistance=off  NormalForceType=SmoothSpringDamper  NormalStiffness=ground.stiffness  NormalStiffnessUnits=N/m  NormalDamping=ground.damping  NormalDampingUnits=N/(m/s)  NormalTransitionRegionWidth=ground.depth/2  NormalTransitionRegionWidthUnits=m  FrictionType=SmoothStickSlip  CoefficientOfStaticFriction=mu_static  CoefficientOfDynamicFriction=mu_kinetic  FrictionalCriticalVelocity=v_thres  FrictionalCriticalVelocityUnits=m/s  SenseContactSignal=off  SensePenetrationDepth=off  SenseNormalVelocity=off  SenseTangentialVelocity=off  SensingForceTorqueDirection=BaseOnFollower  SensingForceTorqueResolutionFrame=ContactFrame  SenseNormalForce=off  SenseNormalForceMagnitude=on  SenseNormalTorque=off  SenseFrictionalForce=off  SenseFrictionalForceMagnitude=on  SenseFrictionalTorque=off  SenseTotalForce=off  SenseTotalTorque=off  SenseContactBaseRotation=off  SenseContactBaseTranslation=off  SenseContactFollowerRotation=off  SenseContactFollowerTranslation=off  ZeroCrossDetectContactStartAndEnd=off
  Upper Leg : Subsystem
  Body : PMIOPort  Side=Left
  Floor : PMIOPort  Tag=PMCPort  Port=2  Side=Right
  sensors : Outport  VectorParamsAs1DForOutWhenUnconnected=off
  contact : Outport  Port=2
  wires:
  Bus Creator/1 -> sensors/1
  Rotary Displacement and Speed Sensor - Knee/1(data) -> Bus Creator/2  "knee"
  Rotary Displacement and Speed Sensor - Hip/1(data) -> Bus Creator/1  "hip"
  Demux/2 -> Knee Actuator/1(torque)  "torque_knee"
  Demux/1 -> Hip Actuator/1(torque)  "torque_hip"
  torque/1 -> Demux/1
  Bus Creator1/1 -> Bus Creator/3  "foot"
  PS-Simulink Converter1/1 -> Bus Creator1/2  "Friction_Force"
  PS-Simulink Converter/1 -> Relational Operator/2, Bus Creator1/1  "Normal_Force"
  Relational Operator/1 -> contact/1
  Constant/1 -> Relational Operator/1
  connections:
  Floor/RConn1 -- Spatial Contact Force/RConn1
  Knee Actuator/RConn3 -- Rotary Displacement and Speed Sensor - Knee/LConn2
  Knee Actuator/RConn2 -- Rotary Displacement and Speed Sensor - Knee/LConn1
  Rotary Displacement and Speed Sensor - Hip/LConn2 -- Hip Actuator/RConn3
  Rotary Displacement and Speed Sensor - Hip/LConn1 -- Hip Actuator/RConn2
  Upper Leg/LConn1 -- Knee Actuator/RConn1
  Upper Leg/RConn1 -- Hip Actuator/LConn1
  Lower Leg/RConn1 -- Knee Actuator/LConn1
  Body/RConn1 -- Hip Actuator/RConn1
  Lower Leg/LConn1 -- Spatial Contact Force/LConn1
  PS-Simulink Converter/LConn1 -- Spatial Contact Force/RConn2
  PS-Simulink Converter1/LConn1 -- Spatial Contact Force/RConn3
  Reference Frame/RConn1 -- Lower Leg/LConn2

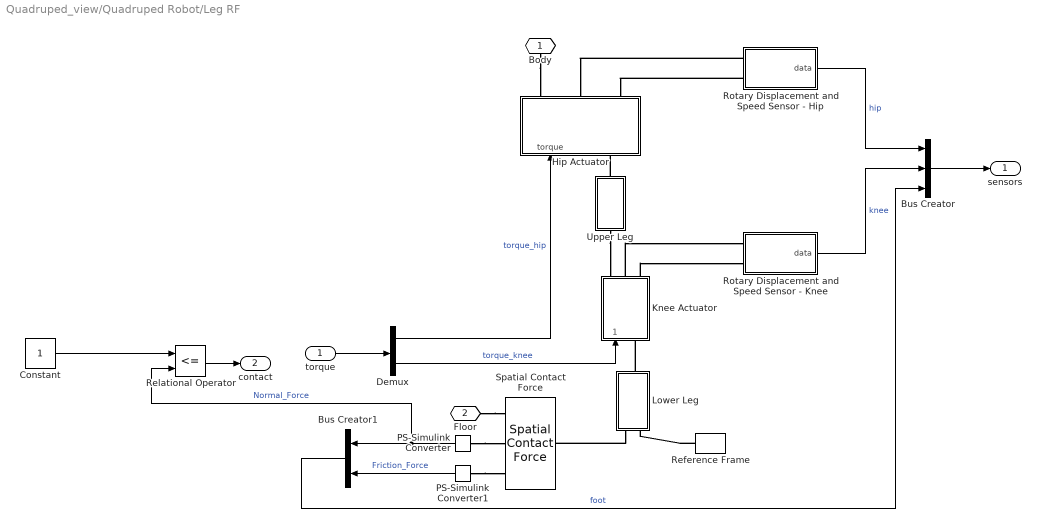
== system Quadruped_view/Quadruped Robot/Leg RF ==
  torque : Inport
  Bus Creator : BusCreator  Inputs=3
  Bus Creator1 : BusCreator  Inputs=2
  Constant : Constant
  Demux : Demux  Outputs=2
  Hip Actuator : Subsystem
  Knee Actuator : Subsystem
  Lower Leg : Subsystem
  PS-Simulink Converter : nesl_utility/PS-Simulink Converter  PhysicalDomain=network_engine_domain  SubClassName=ps_output  LeftPortType=input  RightPortType=output  PseudoPeriodic=off  Frequencies=[]  VectorFormat=1-D array  Unit=inherit  AffineConversion=off
  PS-Simulink Converter1 : nesl_utility/PS-Simulink Converter  PhysicalDomain=network_engine_domain  SubClassName=ps_output  LeftPortType=input  RightPortType=output  PseudoPeriodic=off  Frequencies=[]  VectorFormat=1-D array  Unit=inherit  AffineConversion=off
  Reference Frame : sm_lib/Frames and Transforms/Reference Frame
  Relational Operator : RelationalOperator  Operator=<=  OutDataTypeStr=boolean  RndMeth=Simplest  InputSameDT=off
  Rotary Displacement and Speed Sensor - Hip : Subsystem
  Rotary Displacement and Speed Sensor - Knee : Subsystem
  Spatial Contact Force : sm_lib/Forces and Torques/Spatial Contact Force  SenseSeparationDistance=off  NormalForceType=SmoothSpringDamper  NormalStiffness=ground.stiffness  NormalStiffnessUnits=N/m  NormalDamping=ground.damping  NormalDampingUnits=N/(m/s)  NormalTransitionRegionWidth=ground.depth/2  NormalTransitionRegionWidthUnits=m  FrictionType=SmoothStickSlip  CoefficientOfStaticFriction=mu_static  CoefficientOfDynamicFriction=mu_kinetic  FrictionalCriticalVelocity=v_thres  FrictionalCriticalVelocityUnits=m/s  SenseContactSignal=off  SensePenetrationDepth=off  SenseNormalVelocity=off  SenseTangentialVelocity=off  SensingForceTorqueDirection=BaseOnFollower  SensingForceTorqueResolutionFrame=ContactFrame  SenseNormalForce=off  SenseNormalForceMagnitude=on  SenseNormalTorque=off  SenseFrictionalForce=off  SenseFrictionalForceMagnitude=on  SenseFrictionalTorque=off  SenseTotalForce=off  SenseTotalTorque=off  SenseContactBaseRotation=off  SenseContactBaseTranslation=off  SenseContactFollowerRotation=off  SenseContactFollowerTranslation=off  ZeroCrossDetectContactStartAndEnd=off
  Upper Leg : Subsystem
  Body : PMIOPort  Side=Left
  Floor : PMIOPort  Tag=PMCPort  Port=2  Side=Right
  sensors : Outport  VectorParamsAs1DForOutWhenUnconnected=off
  contact : Outport  Port=2
  wires:
  Bus Creator/1 -> sensors/1
  Rotary Displacement and Speed Sensor - Knee/1(data) -> Bus Creator/2  "knee"
  Rotary Displacement and Speed Sensor - Hip/1(data) -> Bus Creator/1  "hip"
  Demux/2 -> Knee Actuator/1(torque)  "torque_knee"
  Demux/1 -> Hip Actuator/1(torque)  "torque_hip"
  torque/1 -> Demux/1
  PS-Simulink Converter1/1 -> Bus Creator1/2  "Friction_Force"
  PS-Simulink Converter/1 -> Relational Operator/2, Bus Creator1/1  "Normal_Force"
  Bus Creator1/1 -> Bus Creator/3  "foot"
  Constant/1 -> Relational Operator/1
  Relational Operator/1 -> contact/1
  connections:
  Knee Actuator/RConn3 -- Rotary Displacement and Speed Sensor - Knee/LConn2
  Knee Actuator/RConn2 -- Rotary Displacement and Speed Sensor - Knee/LConn1
  Rotary Displacement and Speed Sensor - Hip/LConn2 -- Hip Actuator/RConn3
  Rotary Displacement and Speed Sensor - Hip/LConn1 -- Hip Actuator/RConn2
  Upper Leg/LConn1 -- Knee Actuator/RConn1
  Upper Leg/RConn1 -- Hip Actuator/LConn1
  Lower Leg/RConn1 -- Knee Actuator/LConn1
  Body/RConn1 -- Hip Actuator/RConn1
  Lower Leg/LConn1 -- Spatial Contact Force/LConn1
  Floor/RConn1 -- Spatial Contact Force/RConn1
  PS-Simulink Converter1/LConn1 -- Spatial Contact Force/RConn3
  PS-Simulink Converter/LConn1 -- Spatial Contact Force/RConn2
  Reference Frame/RConn1 -- Lower Leg/LConn2

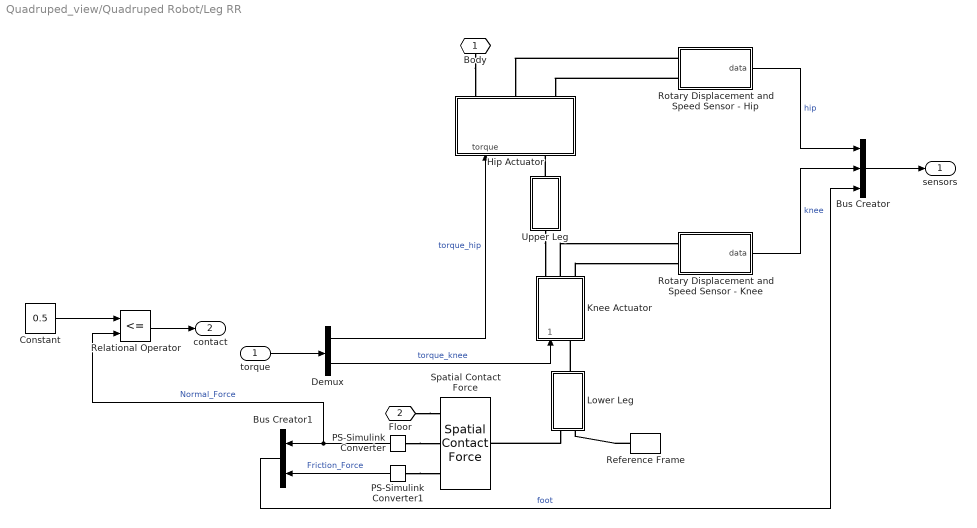
== system Quadruped_view/Quadruped Robot/Leg RR ==
  torque : Inport
  Bus Creator : BusCreator  Inputs=3
  Bus Creator1 : BusCreator  Inputs=2
  Constant : Constant  Value=0.5
  Demux : Demux  Outputs=2
  Hip Actuator : Subsystem
  Knee Actuator : Subsystem
  Lower Leg : Subsystem
  PS-Simulink Converter : nesl_utility/PS-Simulink Converter  PhysicalDomain=network_engine_domain  SubClassName=ps_output  LeftPortType=input  RightPortType=output  PseudoPeriodic=off  Frequencies=[]  VectorFormat=1-D array  Unit=inherit  AffineConversion=off
  PS-Simulink Converter1 : nesl_utility/PS-Simulink Converter  PhysicalDomain=network_engine_domain  SubClassName=ps_output  LeftPortType=input  RightPortType=output  PseudoPeriodic=off  Frequencies=[]  VectorFormat=1-D array  Unit=inherit  AffineConversion=off
  Reference Frame : sm_lib/Frames and Transforms/Reference Frame
  Relational Operator : RelationalOperator  Operator=<=  OutDataTypeStr=boolean  RndMeth=Simplest  InputSameDT=off
  Rotary Displacement and Speed Sensor - Hip : Subsystem
  Rotary Displacement and Speed Sensor - Knee : Subsystem
  Spatial Contact Force : sm_lib/Forces and Torques/Spatial Contact Force  SenseSeparationDistance=off  NormalForceType=SmoothSpringDamper  NormalStiffness=ground.stiffness  NormalStiffnessUnits=N/m  NormalDamping=ground.damping  NormalDampingUnits=N/(m/s)  NormalTransitionRegionWidth=ground.depth/2  NormalTransitionRegionWidthUnits=m  FrictionType=SmoothStickSlip  CoefficientOfStaticFriction=mu_static  CoefficientOfDynamicFriction=mu_kinetic  FrictionalCriticalVelocity=v_thres  FrictionalCriticalVelocityUnits=m/s  SenseContactSignal=off  SensePenetrationDepth=off  SenseNormalVelocity=off  SenseTangentialVelocity=off  SensingForceTorqueDirection=BaseOnFollower  SensingForceTorqueResolutionFrame=ContactFrame  SenseNormalForce=off  SenseNormalForceMagnitude=on  SenseNormalTorque=off  SenseFrictionalForce=off  SenseFrictionalForceMagnitude=on  SenseFrictionalTorque=off  SenseTotalForce=off  SenseTotalTorque=off  SenseContactBaseRotation=off  SenseContactBaseTranslation=off  SenseContactFollowerRotation=off  SenseContactFollowerTranslation=off  ZeroCrossDetectContactStartAndEnd=off
  Upper Leg : Subsystem
  Body : PMIOPort  Side=Left
  Floor : PMIOPort  Tag=PMCPort  Port=2  Side=Right
  sensors : Outport  VectorParamsAs1DForOutWhenUnconnected=off
  contact : Outport  Port=2
  wires:
  Bus Creator/1 -> sensors/1
  Rotary Displacement and Speed Sensor - Knee/1(data) -> Bus Creator/2  "knee"
  Rotary Displacement and Speed Sensor - Hip/1(data) -> Bus Creator/1  "hip"
  Demux/2 -> Knee Actuator/1(torque)  "torque_knee"
  Demux/1 -> Hip Actuator/1(torque)  "torque_hip"
  torque/1 -> Demux/1
  PS-Simulink Converter1/1 -> Bus Creator1/2  "Friction_Force"
  PS-Simulink Converter/1 -> Relational Operator/2, Bus Creator1/1  "Normal_Force"
  Bus Creator1/1 -> Bus Creator/3  "foot"
  Constant/1 -> Relational Operator/1
  Relational Operator/1 -> contact/1
  connections:
  Knee Actuator/RConn3 -- Rotary Displacement and Speed Sensor - Knee/LConn2
  Knee Actuator/RConn2 -- Rotary Displacement and Speed Sensor - Knee/LConn1
  Rotary Displacement and Speed Sensor - Hip/LConn2 -- Hip Actuator/RConn3
  Rotary Displacement and Speed Sensor - Hip/LConn1 -- Hip Actuator/RConn2
  Upper Leg/LConn1 -- Knee Actuator/RConn1
  Upper Leg/RConn1 -- Hip Actuator/LConn1
  Lower Leg/RConn1 -- Knee Actuator/LConn1
  Body/RConn1 -- Hip Actuator/RConn1
  Lower Leg/LConn1 -- Spatial Contact Force/LConn1
  Floor/RConn1 -- Spatial Contact Force/RConn1
  PS-Simulink Converter1/LConn1 -- Spatial Contact Force/RConn3
  PS-Simulink Converter/LConn1 -- Spatial Contact Force/RConn2
  Reference Frame/RConn1 -- Lower Leg/LConn2

== system Quadruped_view/Quadruped Robot/Sensors ==
  Bus Creator : BusCreator  Inputs=7
  From : From  TagVisibility=global
  Leg Sensors : Subsystem
  LowerBody Sensors : Subsystem
  UpperBody Sensors : Subsystem
  Visualization Camera : Subsystem
  CGL : PMIOPort  Side=Left
  CGU : PMIOPort  Port=2  Side=Left
  W : PMIOPort  Port=3  Side=Left
  sensors_out : Outport  VectorParamsAs1DForOutWhenUnconnected=off
  wires:
  UpperBody Sensors/1(UpperBus) -> Bus Creator/2  "Upperbody"
  Bus Creator/1 -> sensors_out/1
  From/1 -> Leg Sensors/1(FL)
  [B] -> Leg Sensors/2(FR)
  [C] -> Leg Sensors/3(RL)
  [D] -> Leg Sensors/4(RR)
  Leg Sensors/1(FLbus) -> Bus Creator/4  "leg_FL"
  Leg Sensors/2(FRbus) -> Bus Creator/5  "leg_FR"
  Leg Sensors/3(RLbus) -> Bus Creator/6  "leg_RL"
  Leg Sensors/4(RRbus) -> Bus Creator/7  "leg_RR"
  LowerBody Sensors/1(LowerBus) -> Bus Creator/3  "Lowerbody"
  UpperBody Sensors/2(direction) -> Bus Creator/1
  connections:
  UpperBody Sensors/LConn2 -- LowerBody Sensors/LConn2 -- W/RConn1
  CGU/RConn1 -- UpperBody Sensors/LConn1 -- Visualization Camera/LConn1
  CGL/RConn1 -- LowerBody Sensors/LConn1

== system Quadruped_view/Quadruped Robot/Subsystem ==
  torques : Inport
  Demux : Demux  Outputs=8
  Mux{,1..3} (4 alike) : Mux  Inputs=2
  RF : Outport  VectorParamsAs1DForOutWhenUnconnected=off
  LF : Outport  Port=2  VectorParamsAs1DForOutWhenUnconnected=off
  RR : Outport  Port=3  VectorParamsAs1DForOutWhenUnconnected=off
  LR : Outport  Port=4  VectorParamsAs1DForOutWhenUnconnected=off
  wires:
  torques/1 -> Demux/1
  Demux/2 -> Mux/2  "torque_knee_FL"
  Demux/3 -> Mux1/1  "torque_hip_FR"
  Demux/4 -> Mux1/2  "torque_knee_FR"
  Demux/5 -> Mux2/1  "torque_hip_RL"
  Demux/6 -> Mux2/2  "torque_knee_RL"
  Demux/8 -> Mux3/2  "torque_knee_RR"
  Demux/7 -> Mux3/1  "torque_hip_RR"
  Mux/1 -> RF/1  "torque_FL"
  Mux1/1 -> LF/1  "torque_FR"
  Mux2/1 -> RR/1  "torque_RL"
  Mux3/1 -> LR/1  "torque_RR"
  Demux/1 -> Mux/1  "torque_hip_FL"
